simulink model "Simulinkexo2"  (R2016a)
settings: Solver=VariableStepAuto  StartTime=0.0  StopTime=250  RelTol=1e-3
settings Model: Creator=KONE MOHAMED  LastModifiedBy=KONE MOHAMED

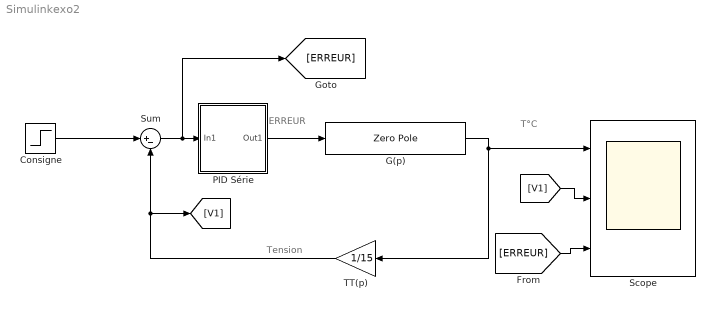
== system Simulinkexo2 ==
  note: Tension
  note: ERREUR
  note: T°C
  Consigne : Step  Time=0  After=80/15  SampleTime=0
  G(p) : ZeroPole  Zeros=[]  Poles=[-1/3.3 -1/3.3 -1/3.3]  Gain=[2/3.3^3]
  "PID Série " : Subsystem
  Scope : Scope  NumInputPorts=3
  Sum : Sum  Inputs=|+-
  TT(p) : Gain  Gain=1/15
  wires:
  Consigne/1 -> Sum/1
  Sum/1 -> "PID Série "/1(In1), [ERREUR]
  G(p)/1 -> TT(p)/1, Scope/1
  TT(p)/1 -> Sum/2, [V1]
  [V1] -> Scope/2
  [ERREUR] -> Scope/3
  "PID Série "/1(Out1) -> G(p)/1

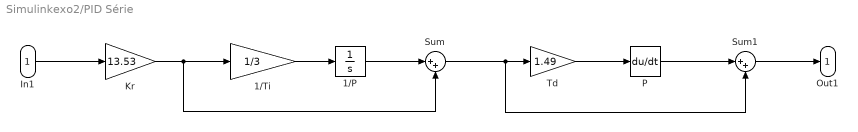
== system Simulinkexo2/PID Série  ==
  In1 : Inport
  "1/P " : Integrator
  "1/Ti " : Gain  Gain=1/3
  "Kr " : Gain  Gain=13.53
  P : Derivative
  Sum : Sum  Inputs=|++
  Sum1 : Sum  Inputs=|++
  Td : Gain  Gain=1.49
  Out1 : Outport
  wires:
  "1/Ti "/1 -> "1/P "/1
  "Kr "/1 -> "1/Ti "/1, Sum/2
  "1/P "/1 -> Sum/1
  In1/1 -> "Kr "/1
  Sum/1 -> Sum1/2, Td/1
  Td/1 -> P/1
  P/1 -> Sum1/1
  Sum1/1 -> Out1/1
